simulink model "VF_Control"  (R2023a)
settings: Solver=ode1  StartTime=0.0  StopTime=Inf  FixedStep=1/16000  RelTol=1e-3
model workspace (MAT data in the model file):
  CLOSE_TO_ZERO = Simulink.Parameter
  CLOSE_TO_ZERO.Value = 1e-05
  CLOSE_TO_ZERO.DataType = 'single'
  CLOSE_TO_ZERO.Complexity = 'real'
  CLOSE_TO_ZERO.Dimensions = [1 1]
  Np = Simulink.Parameter
  Np.Value = 8
  Np.DataType = 'single'
  Np.Complexity = 'real'
  Np.Dimensions = [1 1]
  POLE_NUM = Simulink.Parameter
  POLE_NUM.Value = 8
  POLE_NUM.DataType = 'uint8'
  POLE_NUM.Complexity = 'real'
  POLE_NUM.Dimensions = [1 1]
  SQRT3 = Simulink.Parameter
  SQRT3.Value = 1.7321
  SQRT3.DataType = 'single'
  SQRT3.Complexity = 'real'
  SQRT3.Dimensions = [1 1]
  STEP_SPEED = Simulink.Parameter
  STEP_SPEED.Value = 3
  STEP_SPEED.DataType = 'single'
  STEP_SPEED.Complexity = 'real'
  STEP_SPEED.Dimensions = [1 1]
undefined symbols (not defined in the file): TS
libraries: mcbplantlib x1, simulink x1, autolibpmsmexterior x1
settings Model: Creator=hyowi  LastModifiedBy=hyowi
settings DataIOCC: SaveOutput=off  SignalLogging=off  DSMLogging=off  SaveTime=off  ReturnWorkspaceOutputs=off

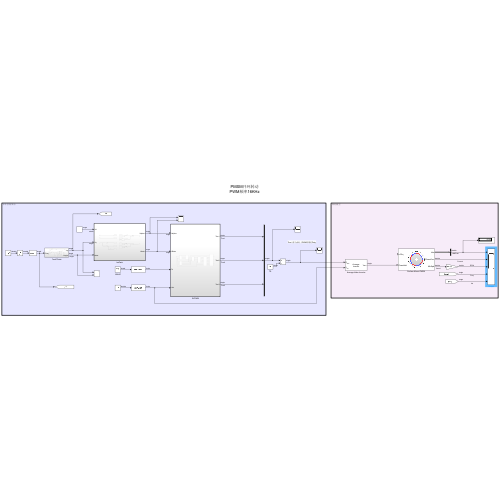
[thumbnail: Simulink's stored preview of the top-level diagram]
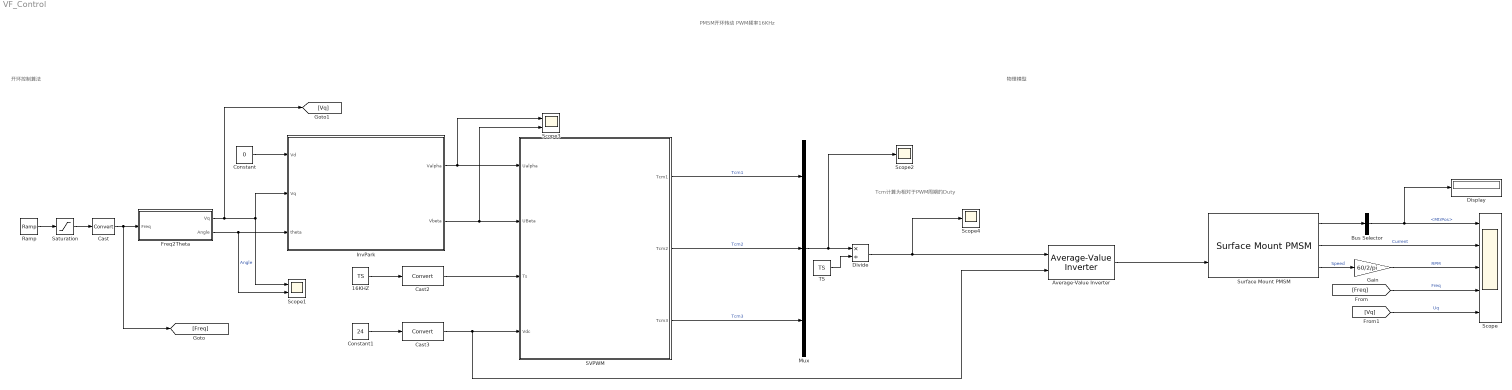
== system VF_Control ==
  note: 物理模型
  note: 开环控制算法
  note: Tcm计算为相对于PWM周期的Duty
  note: PMSM开环转动
      | PWM频率16KHz
  16KHZ : Constant  Value=TS
  Average-Value Inverter : mcbplantlib/Average-Value Inverter
      settings: LibrarySourceBlock=mcblib/Electrical Systems/Inverters/Average-Value Inverter
  Bus Selector : BusSelector  OutputSignals=MtrPos
  Cast : DataTypeConversion  SaturateOnIntegerOverflow=off  RndMeth=Floor
  Cast2 : DataTypeConversion  SaturateOnIntegerOverflow=off  RndMeth=Floor
  Cast3 : DataTypeConversion  SaturateOnIntegerOverflow=off  RndMeth=Floor
  Constant : Constant  Value=0  OutDataTypeStr=single
  Constant1 : Constant  Value=24  SampleTime=-1
  Display : Display
  Divide : Product  Inputs=*/
  Freq2Theta : Subsystem
  Gain : Gain  Gain=60/2/pi
  InvPark : Subsystem  TreatAsAtomicUnit=on
  Mux : Mux  Inputs=3
  Ramp : simulink/Sources/Ramp  slope=12  start=2  InitialOutput=15
  SVPWM : Subsystem  TreatAsAtomicUnit=on
  Saturation : Saturate  UpperLimit=400
  Scope : Scope  NumInputPorts=5
  Scope1 : Scope  NumInputPorts=2
  Scope2 : Scope
  Scope3 : Scope  NumInputPorts=2
  Scope4 : Scope
  Surface Mount PMSM : autolibpmsmexterior/Surface Mount PMSM  port_config=Torque  sim_type=Discrete  Ts=1/16000  FilePath=E:\Sandbox\Bauto\Work\surfacepmsm_motordata.m  P=8  Rs=1.02  Ldq_=0.59e-3  KConstText=Permanent flux linkage constant (lambda_pm):  lambda_pm=0.01194  Ke=159.9771  Kt=1.323  mechanical=[0.0047, 4.924e-4, 0]  idq0=[0 0]  theta_init=0  omega_init=0  KConst=0.01194  lambda_pm_calc=0.01194  RefBlkName='autolibpmsmexterior/Surface Mount PMSM'  aMode=1  Ldq="[0.0003752   0.0003752]"
      settings: LibrarySourceBlock=autolibemachines/Surface Mount PMSM
  TS : Constant  Value=TS
  wires:
  16KHZ/1 -> Cast2/1
  Constant1/1 -> Cast3/1
  Cast2/1 -> SVPWM/3(Ts)
  Cast3/1 -> Average-Value Inverter/2, SVPWM/4(Vdc)
  InvPark/1(Valpha) -> Scope3/1, SVPWM/1(Ualpha)
  InvPark/2(Vbeta) -> Scope3/2, SVPWM/2(UBeta)
  Mux/1 -> Scope2/1, Divide/1
  TS/1 -> Divide/2
  Average-Value Inverter/1 -> Surface Mount PMSM/2
  Surface Mount PMSM/2 -> Scope/2  "Current"
  Constant/1 -> InvPark/1(Vd)
  Saturation/1 -> Cast/1
  Freq2Theta/2(Angle) -> Scope1/2, InvPark/3(theta)  "Angle"
  Ramp/1 -> Saturation/1
  Cast/1 -> [Freq], Freq2Theta/1(Freq)
  Divide/1 -> Scope4/1, Average-Value Inverter/1
  Surface Mount PMSM/3 -> Gain/1  "Speed"
  Gain/1 -> Scope/3  "RPM"
  [Freq] -> Scope/4  "Freq"
  [Vq] -> Scope/5  "Uq"
  Freq2Theta/1(Vq) -> [Vq], InvPark/2(Vq), Scope1/1
  Surface Mount PMSM/1 -> Bus Selector/1
  Bus Selector/1 -> Display/1, Scope/1  "<MtrPos>"
  SVPWM/1(Tcm1) -> Mux/1  "Tcm1"
  SVPWM/2(Tcm2) -> Mux/2  "Tcm2"
  SVPWM/3(Tcm3) -> Mux/3  "Tcm3"

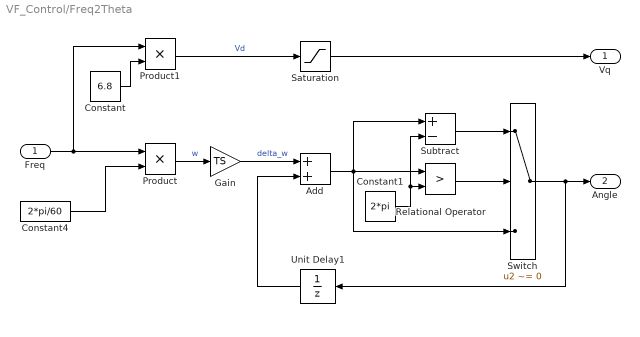
== system VF_Control/Freq2Theta ==
  Freq : Inport
  Add : Sum
  Constant : Constant  Value=6.8  OutDataTypeStr=single
  Constant1 : Constant  Value=2*pi  OutDataTypeStr=single
  Constant4 : Constant  Value=2*pi/60  OutDataTypeStr=single
  Gain : Gain  Gain=TS
  Product : Product
  Product1 : Product
  Relational Operator : RelationalOperator  Operator=>  OutDataTypeStr=boolean  RndMeth=Simplest  InputSameDT=off
  Saturation : Saturate  UpperLimit=24/sqrt(3)  LowerLimit=2
  Subtract : Sum  Inputs=+-
  Switch : Switch  Criteria=u2 ~= 0  SaturateOnIntegerOverflow=off  InputSameDT=off
  Unit Delay1 : UnitDelay  SampleTime=-1  HasFrameUpgradeWarning=on
  Vq : Outport
  Angle : Outport  Port=2
  wires:
  Product/1 -> Gain/1  "w"
  Constant4/1 -> Product/2
  Freq/1 -> Product1/1, Product/1
  Unit Delay1/1 -> Add/2
  Constant/1 -> Product1/2
  Product1/1 -> Saturation/1  "Vd"
  Saturation/1 -> Vq/1
  Gain/1 -> Add/1  "delta_w"
  Switch/1 -> Unit Delay1/1, Angle/1
  Relational Operator/1 -> Switch/2
  Add/1 -> Subtract/1, Switch/3, Relational Operator/1
  Constant1/1 -> Subtract/2, Relational Operator/2
  Subtract/1 -> Switch/1

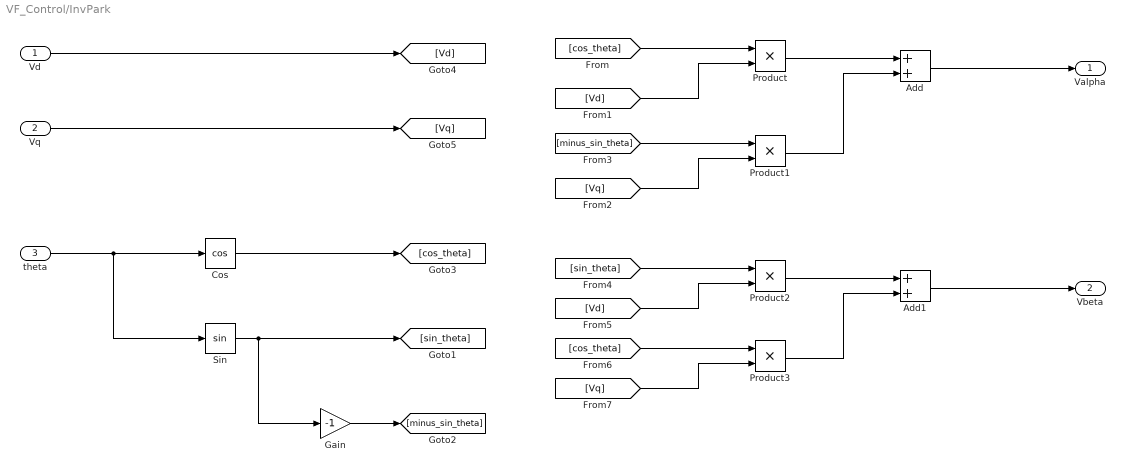
== system VF_Control/InvPark ==
  Vd : Inport  OutDataTypeStr=single
  Vq : Inport  Port=2  OutDataTypeStr=single
  theta : Inport  Port=3
  Add : Sum
  Add1 : Sum
  Cos : Trigonometry  Operator=cos
  Gain : Gain  Gain=-1
  Product{,1..3} (4 alike) : Product
  Sin : Trigonometry
  Valpha : Outport
  Vbeta : Outport  Port=2
  wires:
  [cos_theta] -> Product3/1
  Add1/1 -> Vbeta/1
  [Vq] -> Product1/2
  theta/1 -> Sin/1, Cos/1
  Sin/1 -> Gain/1, [sin_theta]
  Product/1 -> Add/1
  [Vd] -> Product2/2
  Product3/1 -> Add1/2
  [Vq] -> Product3/2
  [cos_theta] -> Product/1
  Product2/1 -> Add1/1
  Gain/1 -> [minus_sin_theta]
  Vd/1 -> [Vd]
  Add/1 -> Valpha/1
  Vq/1 -> [Vq]
  Cos/1 -> [cos_theta]
  [Vd] -> Product/2
  [minus_sin_theta] -> Product1/1
  [sin_theta] -> Product2/1
  Product1/1 -> Add/2

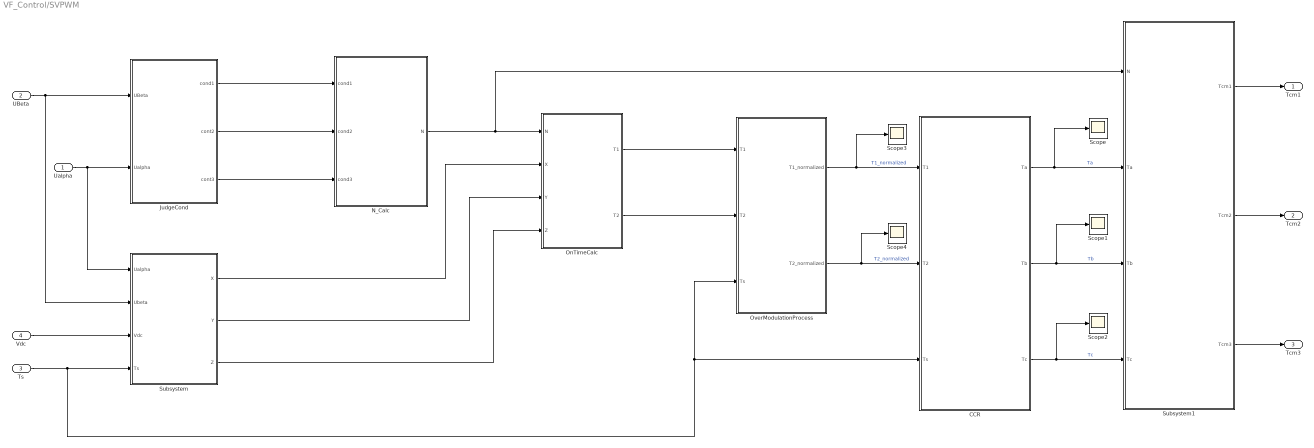
== system VF_Control/SVPWM ==
  Ualpha : Inport  OutDataTypeStr=single
  UBeta : Inport  Port=2  OutDataTypeStr=single
  Ts : Inport  Port=3
  Vdc : Inport  Port=4
  CCR : Subsystem  TreatAsAtomicUnit=on
  JudgeCond : Subsystem  TreatAsAtomicUnit=on
  N_Calc : Subsystem  TreatAsAtomicUnit=on
  OnTimeCalc : Subsystem  TreatAsAtomicUnit=on
  OverModulationProcess : Subsystem  TreatAsAtomicUnit=on
  Scope{,1..4} (5 alike) : Scope
  Subsystem : Subsystem  TreatAsAtomicUnit=on
  Subsystem1 : Subsystem  TreatAsAtomicUnit=on
  Tcm1 : Outport
  Tcm2 : Outport  Port=2
  Tcm3 : Outport  Port=3
  wires:
  Vdc/1 -> Subsystem/3(Vdc)
  JudgeCond/1(cond1) -> N_Calc/1(cond1)
  OnTimeCalc/1(T1) -> OverModulationProcess/1(T1)
  OnTimeCalc/2(T2) -> OverModulationProcess/2(T2)
  Subsystem/2(Y) -> OnTimeCalc/3(Y)
  Subsystem/3(Z) -> OnTimeCalc/4(Z)
  Ts/1 -> OverModulationProcess/3(Ts), CCR/3(Ts), Subsystem/4(Ts)
  OverModulationProcess/2(T2_normalized) -> Scope4/1, CCR/2(T2)  "T2_normalized"
  OverModulationProcess/1(T1_normalized) -> Scope3/1, CCR/1(T1)  "T1_normalized"
  Subsystem/1(X) -> OnTimeCalc/2(X)
  Ualpha/1 -> Subsystem/1(Ualpha), JudgeCond/2(Ualpha)
  UBeta/1 -> Subsystem/2(Ubeta), JudgeCond/1(UBeta)
  Subsystem1/1(Tcm1) -> Tcm1/1
  Subsystem1/2(Tcm2) -> Tcm2/1
  Subsystem1/3(Tcm3) -> Tcm3/1
  CCR/1(Ta) -> Scope/1, Subsystem1/2(Ta)  "Ta"
  CCR/2(Tb) -> Scope1/1, Subsystem1/3(Tb)  "Tb"
  CCR/3(Tc) -> Scope2/1, Subsystem1/4(Tc)  "Tc"
  JudgeCond/2(cont2) -> N_Calc/2(cond2)
  JudgeCond/3(cont3) -> N_Calc/3(cond3)
  N_Calc/1(N) -> Subsystem1/1(N), OnTimeCalc/1(N)

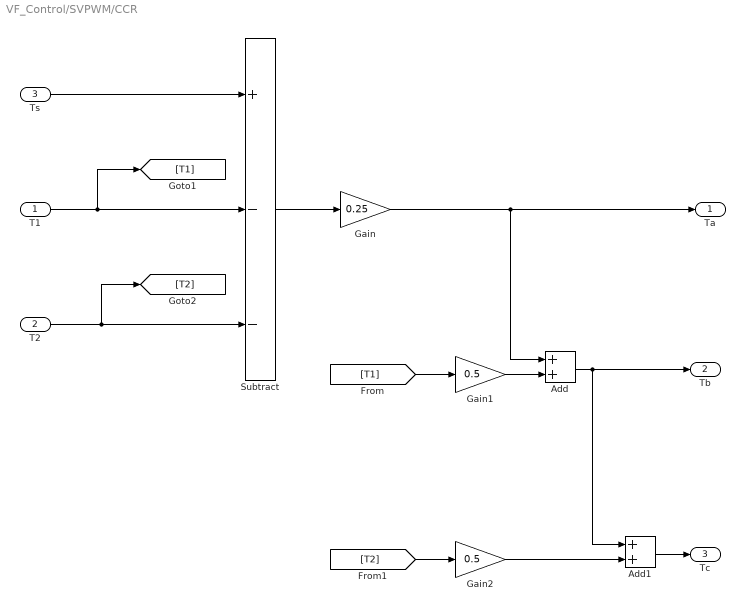
== system VF_Control/SVPWM/CCR ==
  T1 : Inport
  T2 : Inport  Port=2
  Ts : Inport  Port=3
  Add : Sum
  Add1 : Sum
  Gain : Gain  Gain=0.25  OutDataTypeStr=Inherit: Same as input
  Gain1 : Gain  Gain=0.5  OutDataTypeStr=Inherit: Same as input
  Gain2 : Gain  Gain=0.5  OutDataTypeStr=Inherit: Same as input
  Subtract : Sum  Inputs=+--
  Ta : Outport
  Tb : Outport  Port=2
  Tc : Outport  Port=3
  wires:
  Subtract/1 -> Gain/1
  Add/1 -> Tb/1, Add1/1
  Gain/1 -> Ta/1, Add/1
  [T1] -> Gain1/1
  T1/1 -> [T1], Subtract/2
  [T2] -> Gain2/1
  T2/1 -> [T2], Subtract/3
  Add1/1 -> Tc/1
  Ts/1 -> Subtract/1
  Gain1/1 -> Add/2
  Gain2/1 -> Add1/2

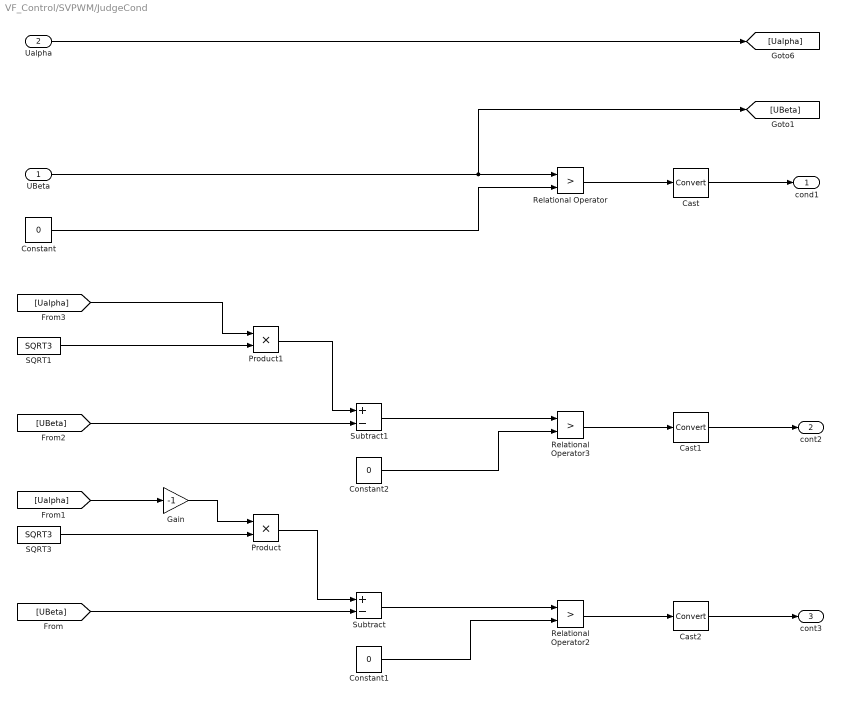
== system VF_Control/SVPWM/JudgeCond ==
  UBeta : Inport  OutDataTypeStr=single
  Ualpha : Inport  Port=2  OutDataTypeStr=single
  Cast : DataTypeConversion  SaturateOnIntegerOverflow=off  RndMeth=Floor
  Cast1 : DataTypeConversion  SaturateOnIntegerOverflow=off  RndMeth=Floor
  Cast2 : DataTypeConversion  SaturateOnIntegerOverflow=off  RndMeth=Floor
  Constant : Constant  Value=0  OutDataTypeStr=single
  Constant1 : Constant  Value=0  OutDataTypeStr=single
  Constant2 : Constant  Value=0  OutDataTypeStr=single
  Gain : Gain  Gain=-1
  Product : Product
  Product1 : Product
  Relational Operator : RelationalOperator  Operator=>  OutDataTypeStr=boolean  RndMeth=Simplest  InputSameDT=off
  Relational Operator2 : RelationalOperator  Operator=>  OutDataTypeStr=boolean  RndMeth=Simplest  InputSameDT=off
  Relational Operator3 : RelationalOperator  Operator=>  OutDataTypeStr=boolean  RndMeth=Simplest  InputSameDT=off
  SQRT1 : Constant  Value=SQRT3  OutDataTypeStr=single
  SQRT3 : Constant  Value=SQRT3  OutDataTypeStr=single
  Subtract : Sum  Inputs=+-
  Subtract1 : Sum  Inputs=+-
  cond1 : Outport  OutDataTypeStr=uint8
  cont2 : Outport  Port=2  OutDataTypeStr=uint8
  cont3 : Outport  Port=3  OutDataTypeStr=uint8
  wires:
  UBeta/1 -> Relational Operator/1, [UBeta]
  Relational Operator/1 -> Cast/1
  Constant/1 -> Relational Operator/2
  Relational Operator2/1 -> Cast2/1
  Relational Operator3/1 -> Cast1/1
  Ualpha/1 -> [Ualpha]
  Cast/1 -> cond1/1
  Cast1/1 -> cont2/1
  Cast2/1 -> cont3/1
  Product/1 -> Subtract/1
  SQRT3/1 -> Product/2
  Subtract/1 -> Relational Operator2/1
  Constant1/1 -> Relational Operator2/2
  SQRT1/1 -> Product1/2
  Subtract1/1 -> Relational Operator3/1
  Product1/1 -> Subtract1/1
  Constant2/1 -> Relational Operator3/2
  [UBeta] -> Subtract/2
  [Ualpha] -> Gain/1
  [UBeta] -> Subtract1/2
  [Ualpha] -> Product1/1
  Gain/1 -> Product/1

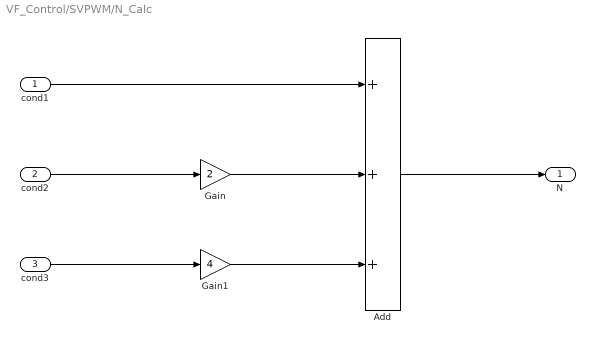
== system VF_Control/SVPWM/N_Calc ==
  cond1 : Inport  OutDataTypeStr=uint8
  cond2 : Inport  Port=2  OutDataTypeStr=uint8
  cond3 : Inport  Port=3  OutDataTypeStr=uint8
  Add : Sum  Inputs=+++
  Gain : Gain  Gain=2  OutDataTypeStr=Inherit: Same as input
  Gain1 : Gain  Gain=4  OutDataTypeStr=Inherit: Same as input
  N : Outport
  wires:
  cond3/1 -> Gain1/1
  cond1/1 -> Add/1
  Add/1 -> N/1
  cond2/1 -> Gain/1
  Gain1/1 -> Add/3
  Gain/1 -> Add/2

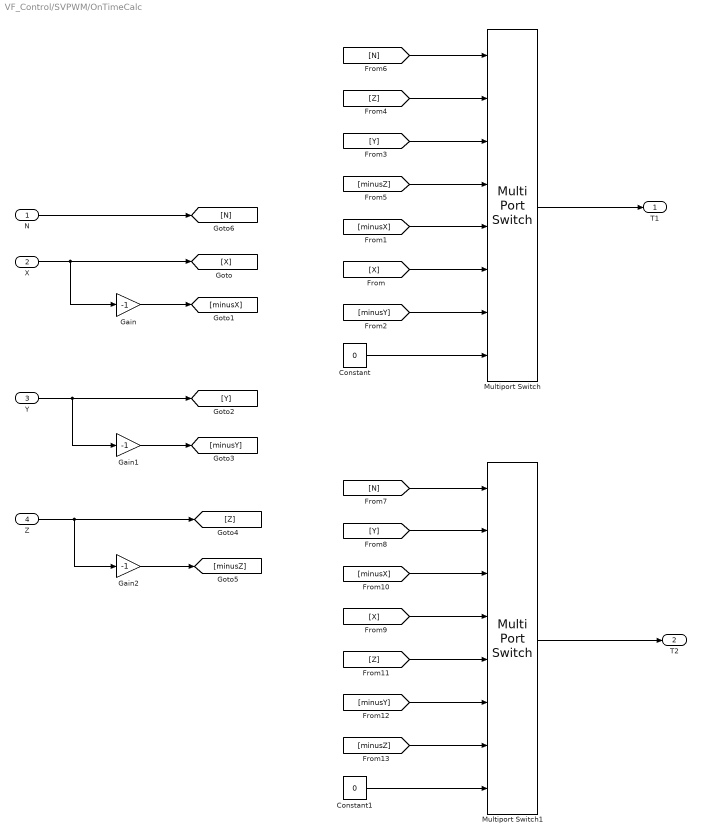
== system VF_Control/SVPWM/OnTimeCalc ==
  N : Inport
  X : Inport  Port=2  OutDataTypeStr=single
  Y : Inport  Port=3  OutDataTypeStr=single
  Z : Inport  Port=4  OutDataTypeStr=single
  Constant : Constant  Value=0  OutDataTypeStr=single
  Constant1 : Constant  Value=0  OutDataTypeStr=single
  Gain : Gain  Gain=-1  OutDataTypeStr=single
  Gain1 : Gain  Gain=-1  OutDataTypeStr=single
  Gain2 : Gain  Gain=-1  OutDataTypeStr=single
  Multiport Switch : MultiPortSwitch  Inputs=7  DiagnosticForDefault=Warning  SaturateOnIntegerOverflow=off  InputSameDT=off
  Multiport Switch1 : MultiPortSwitch  Inputs=7  DiagnosticForDefault=Warning  SaturateOnIntegerOverflow=off  InputSameDT=off
  T1 : Outport
  T2 : Outport  Port=2
  wires:
  [N] -> Multiport Switch/1
  [minusZ] -> Multiport Switch1/7
  [minusY] -> Multiport Switch1/6
  Multiport Switch1/1 -> T2/1
  [minusX] -> Multiport Switch/5
  Constant/1 -> Multiport Switch/8
  Z/1 -> Gain2/1, [Z]
  X/1 -> Gain/1, [X]
  [Y] -> Multiport Switch1/2
  [Z] -> Multiport Switch1/5
  [minusZ] -> Multiport Switch/4
  [Y] -> Multiport Switch/3
  Y/1 -> Gain1/1, [Y]
  [minusX] -> Multiport Switch1/3
  Multiport Switch/1 -> T1/1
  Gain1/1 -> [minusY]
  Gain2/1 -> [minusZ]
  [X] -> Multiport Switch1/4
  [X] -> Multiport Switch/6
  Gain/1 -> [minusX]
  Constant1/1 -> Multiport Switch1/8
  [Z] -> Multiport Switch/2
  [N] -> Multiport Switch1/1
  [minusY] -> Multiport Switch/7
  N/1 -> [N]

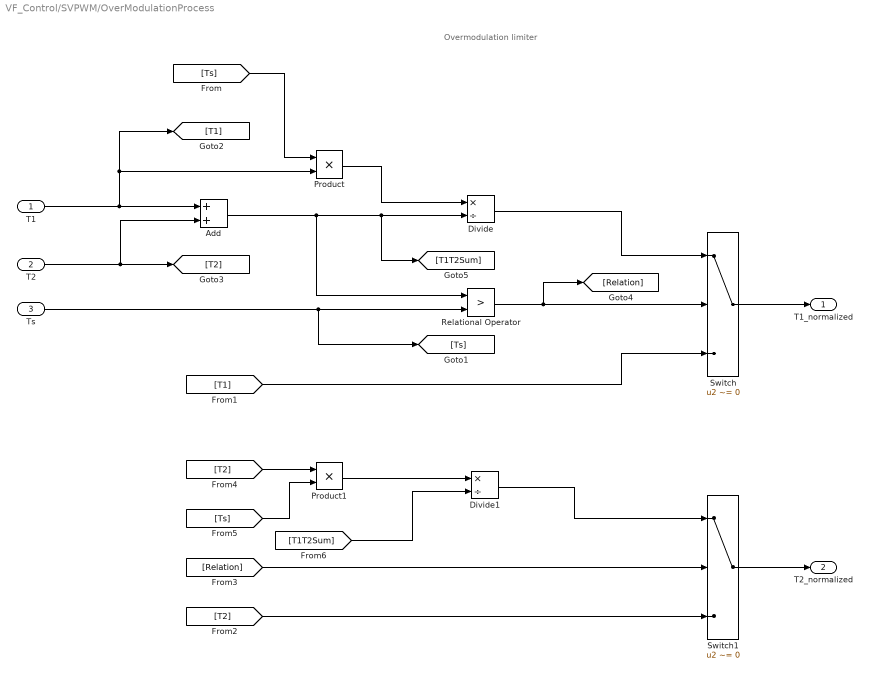
== system VF_Control/SVPWM/OverModulationProcess ==
  note: Overmodulation limiter
  T1 : Inport
  T2 : Inport  Port=2
  Ts : Inport  Port=3
  Add : Sum
  Divide : Product  Inputs=*/
  Divide1 : Product  Inputs=*/
  Product : Product
  Product1 : Product
  Relational Operator : RelationalOperator  Operator=>  OutDataTypeStr=boolean  RndMeth=Simplest  InputSameDT=off
  Switch : Switch  Criteria=u2 ~= 0  SaturateOnIntegerOverflow=off  InputSameDT=off
  Switch1 : Switch  Criteria=u2 ~= 0  SaturateOnIntegerOverflow=off  InputSameDT=off
  T1_normalized : Outport
  T2_normalized : Outport  Port=2
  wires:
  Add/1 -> [T1T2Sum], Divide/2, Relational Operator/1
  [Ts] -> Product/1
  T1/1 -> Add/1, Product/2, [T1]
  Ts/1 -> Relational Operator/2, [Ts]
  Relational Operator/1 -> [Relation], Switch/2
  [T1] -> Switch/3
  Product/1 -> Divide/1
  Switch/1 -> T1_normalized/1
  Divide/1 -> Switch/1
  T2/1 -> [T2], Add/2
  [Relation] -> Switch1/2
  [T2] -> Switch1/3
  Divide1/1 -> Switch1/1
  Switch1/1 -> T2_normalized/1
  [T2] -> Product1/1
  [Ts] -> Product1/2
  Product1/1 -> Divide1/1
  [T1T2Sum] -> Divide1/2

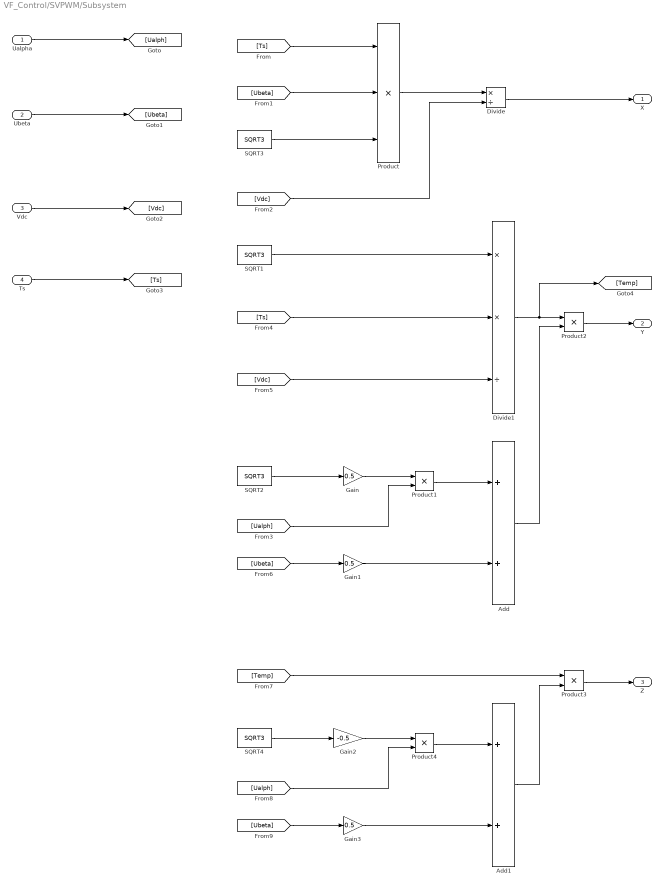
== system VF_Control/SVPWM/Subsystem ==
  Ualpha : Inport
  Ubeta : Inport  Port=2
  Vdc : Inport  Port=3
  Ts : Inport  Port=4
  Add : Sum
  Add1 : Sum
  Divide : Product  Inputs=*/
  Divide1 : Product  Inputs=**/
  Gain : Gain  Gain=0.5
  Gain1 : Gain  Gain=0.5
  Gain2 : Gain  Gain=-0.5
  Gain3 : Gain  Gain=0.5
  Product : Product  Inputs=3
  Product{1..4} (4 alike) : Product
  SQRT{1..4} (4 alike) : Constant  Value=SQRT3  OutDataTypeStr=single
  X : Outport
  Y : Outport  Port=2
  Z : Outport  Port=3
  wires:
  Ualpha/1 -> [Ualph]
  Ubeta/1 -> [Ubeta]
  Vdc/1 -> [Vdc]
  Ts/1 -> [Ts]
  [Ts] -> Product/1
  [Ubeta] -> Product/2
  SQRT3/1 -> Product/3
  Product/1 -> Divide/1
  Divide/1 -> X/1
  [Vdc] -> Divide/2
  SQRT1/1 -> Divide1/1
  [Ts] -> Divide1/2
  [Vdc] -> Divide1/3
  Product1/1 -> Add/1
  Gain/1 -> Product1/1
  SQRT2/1 -> Gain/1
  [Ualph] -> Product1/2
  [Ubeta] -> Gain1/1
  Gain1/1 -> Add/2
  Divide1/1 -> [Temp], Product2/1
  Add/1 -> Product2/2
  Product2/1 -> Y/1
  [Temp] -> Product3/1
  Product3/1 -> Z/1
  [Ualph] -> Product4/2
  Gain2/1 -> Product4/1
  [Ubeta] -> Gain3/1
  SQRT4/1 -> Gain2/1
  Product4/1 -> Add1/1
  Gain3/1 -> Add1/2
  Add1/1 -> Product3/2

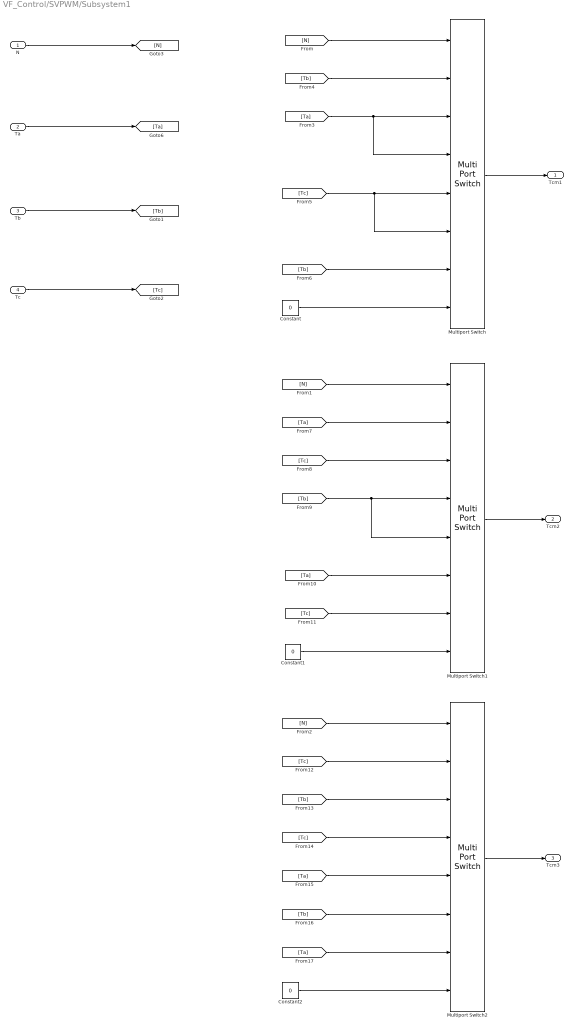
== system VF_Control/SVPWM/Subsystem1 ==
  N : Inport
  Ta : Inport  Port=2
  Tb : Inport  Port=3
  Tc : Inport  Port=4
  Constant : Constant  Value=0  OutDataTypeStr=single
  Constant1 : Constant  Value=0  OutDataTypeStr=single
  Constant2 : Constant  Value=0  OutDataTypeStr=single
  Multiport Switch : MultiPortSwitch  Inputs=7  DiagnosticForDefault=Warning  SaturateOnIntegerOverflow=off  InputSameDT=off
  Multiport Switch1 : MultiPortSwitch  Inputs=7  DiagnosticForDefault=Warning  SaturateOnIntegerOverflow=off  InputSameDT=off
  Multiport Switch2 : MultiPortSwitch  Inputs=7  DiagnosticForDefault=Warning  SaturateOnIntegerOverflow=off  InputSameDT=off
  Tcm1 : Outport
  Tcm2 : Outport  Port=2
  Tcm3 : Outport  Port=3
  wires:
  Ta/1 -> [Ta]
  Tb/1 -> [Tb]
  Tc/1 -> [Tc]
  N/1 -> [N]
  Multiport Switch/1 -> Tcm1/1
  Multiport Switch1/1 -> Tcm2/1
  Multiport Switch2/1 -> Tcm3/1
  [N] -> Multiport Switch/1
  [N] -> Multiport Switch1/1
  [N] -> Multiport Switch2/1
  [Tb] -> Multiport Switch/2
  [Ta] -> Multiport Switch/4, Multiport Switch/3
  [Tc] -> Multiport Switch/6, Multiport Switch/5
  [Tb] -> Multiport Switch/7
  Constant/1 -> Multiport Switch/8
  [Ta] -> Multiport Switch1/2
  [Tc] -> Multiport Switch1/3
  [Tb] -> Multiport Switch1/5, Multiport Switch1/4
  [Ta] -> Multiport Switch1/6
  [Tc] -> Multiport Switch1/7
  Constant1/1 -> Multiport Switch1/8
  [Tc] -> Multiport Switch2/2
  [Tb] -> Multiport Switch2/3
  [Tc] -> Multiport Switch2/4
  [Ta] -> Multiport Switch2/5
  [Tb] -> Multiport Switch2/6
  [Ta] -> Multiport Switch2/7
  Constant2/1 -> Multiport Switch2/8
